simulink model "tarea7"  (R2026b)
settings: Solver=VariableStepAuto  StopTime=2
settings Model: LastModifiedBy=rosa georgina

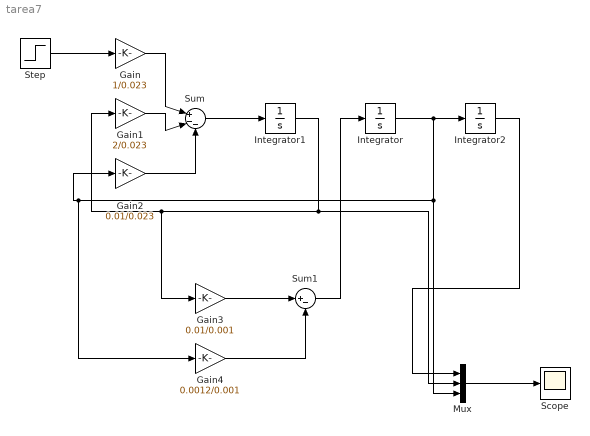
== system tarea7 ==
  Gain : Gain  Gain=1/0.023
  Gain1 : Gain  Gain=2/0.023
  Gain2 : Gain  Gain=0.01/0.023
  Gain3 : Gain  Gain=0.01/0.001
  Gain4 : Gain  Gain=0.0012/0.001
  Integrator : Integrator
  Integrator1 : Integrator
  Integrator2 : Integrator
  Mux : Mux  Inputs=3
  Scope : Scope
      settings: ActiveDisplayYMinimum=-7.5327052468492708  ActiveDisplayYMaximum=67.794347221643449
  Step : Step  Time=0  FinalValue=12  SampleTime=0
  Sum : Sum  Inputs=|+--
  Sum1 : Sum  Inputs=|+-
  wires:
  Step/1 -> Gain/1
  Gain/1 -> Sum/1
  Gain1/1 -> Sum/2
  Gain2/1 -> Sum/3
  Sum/1 -> Integrator1/1
  Gain3/1 -> Sum1/1
  Gain4/1 -> Sum1/2
  Sum1/1 -> Integrator/1
  Integrator/1 -> Gain4/1, Gain2/1, Mux/3, Integrator2/1
  Integrator1/1 -> Mux/2, Gain3/1, Gain1/1
  Mux/1 -> Scope/1
  Integrator2/1 -> Mux/1
